simulink model "Guidance_MVP_AI"  (R2026b)
settings: Solver=ode4  StopTime=90  FixedStep=0.005
settings Model: DataDictionary=QuadInterfaces_AI.sldd  Creator=JonathanTee  LastModifiedBy=JonathanTee

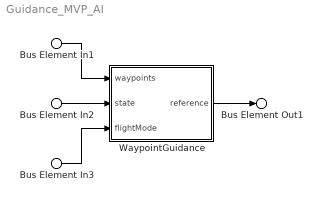
== system Guidance_MVP_AI ==
  Bus Element In1 : Inport  PortName=WaypointTargets
  Bus Element In2 : Inport  Port=2  PortName=VehicleState
  Bus Element In3 : Inport  Port=3  PortName=FlightMode
  WaypointGuidance : MATLAB Function  TreatAsAtomicUnit=on
  Bus Element Out1 : Outport  PortName=PositionReference
  wires:
  WaypointGuidance/1(reference) -> Bus Element Out1/1
  Bus Element In3/1 -> WaypointGuidance/3(flightMode)
  Bus Element In2/1 -> WaypointGuidance/2(state)
  Bus Element In1/1 -> WaypointGuidance/1(waypoints)

== matlab function Guidance_MVP_AI/WaypointGuidance ==
  settings: updateMethod=DISCRETE  sampleTime=MVP.SampleTime
  data: waypoints input Bus: WaypointTargets_IF; reference output Bus: PositionReference_IF; state input Bus: VehicleState_IF; flightMode input Bus: FlightMode_IF
function reference=guidance(waypoints,state,flightMode)
%#codegen
reference=stage02_guidance(waypoints,state,flightMode);
end
